simulink model "hdlcoder_addwc_eml"  (R2026a)
settings: Solver=FixedStepDiscrete  StopTime=10  FixedStep=1
settings Model: Creator=The MathWorks, Inc.  LastModifiedBy=The MathWorks, Inc.
settings OptimizationCC: ConditionallyExecuteInputs=off  InitFltsAndDblsToZero=on
settings DebuggingCC: AlgebraicLoopMsg=error  UnderspecifiedInitializationDetection=Classic  MultiTaskDSMMsg=warning  MultiTaskCondExecSysMsg=none  SingleTaskRateTransMsg=error
settings HardwareCC: ProdHWDeviceType=ASIC/FPGA
settings GRTTargetCC: TargetFcnLib=ansi_tfl_tmw_new.mat  CombineOutputUpdateFcns=off  GRTInterface=on

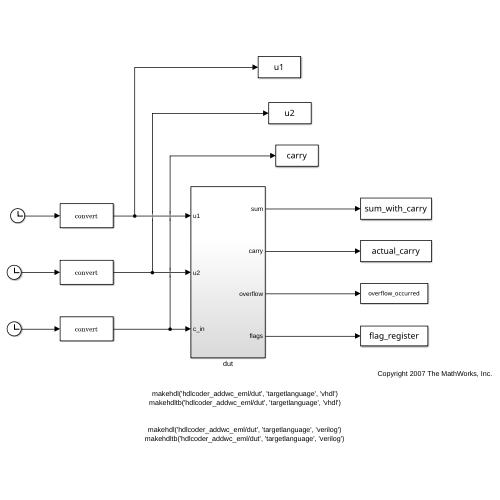
[thumbnail: Simulink's stored preview of the top-level diagram]
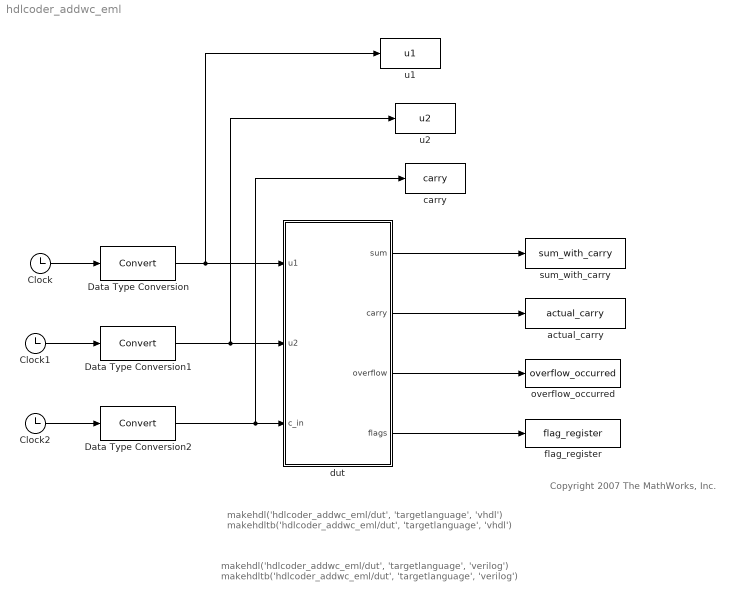
== system hdlcoder_addwc_eml ==
  note: Copyright 2007 The MathWorks, Inc.
  note: makehdl('hdlcoder_addwc_eml/dut', 'targetlanguage', 'vhdl')
      | makehdltb('hdlcoder_addwc_eml/dut', 'targetlanguage', 'vhdl')
  note: makehdl('hdlcoder_addwc_eml/dut', 'targetlanguage', 'verilog')
      | makehdltb('hdlcoder_addwc_eml/dut', 'targetlanguage', 'verilog')
  Clock : Clock
  Clock1 : Clock
  Clock2 : Clock
  Data Type Conversion : DataTypeConversion  SaturateOnIntegerOverflow=off  RndMeth=Floor
  Data Type Conversion1 : DataTypeConversion  SaturateOnIntegerOverflow=off  RndMeth=Floor
  Data Type Conversion2 : DataTypeConversion  SaturateOnIntegerOverflow=off  RndMeth=Floor
  actual_carry : ToWorkspace  VariableName=actual_carry  SampleTime=-1
  carry : ToWorkspace  VariableName=carry  SampleTime=-1
  dut : Subsystem
  flag_register : ToWorkspace  VariableName=flag_register  SampleTime=-1
  overflow_occurred : ToWorkspace  VariableName=overflow_occurred  SampleTime=-1
  sum_with_carry : ToWorkspace  VariableName=sum_with_carry  SampleTime=-1
  u1 : ToWorkspace  VariableName=u1  SampleTime=-1
  u2 : ToWorkspace  VariableName=u2  SampleTime=-1
  wires:
  Clock/1 -> Data Type Conversion/1
  Clock1/1 -> Data Type Conversion1/1
  Clock2/1 -> Data Type Conversion2/1
  Data Type Conversion/1 -> dut/1(u1), u1/1
  Data Type Conversion1/1 -> dut/2(u2), u2/1
  Data Type Conversion2/1 -> dut/3(c_in), carry/1
  dut/1(sum) -> sum_with_carry/1
  dut/2(carry) -> actual_carry/1
  dut/3(overflow) -> overflow_occurred/1
  dut/4(flags) -> flag_register/1

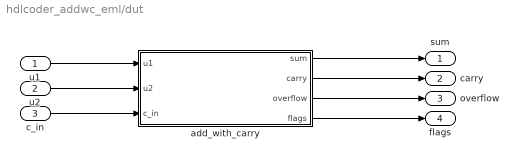
== system hdlcoder_addwc_eml/dut ==
  u1 : Inport
  u2 : Inport  Port=2
  c_in : Inport  Port=3
  add_with_carry : MATLAB Function  TreatAsAtomicUnit=on
  sum : Outport
  carry : Outport  Port=2
  overflow : Outport  Port=3
  flags : Outport  Port=4
  wires:
  add_with_carry/4(flags) -> flags/1
  c_in/1 -> add_with_carry/3(c_in)
  add_with_carry/3(overflow) -> overflow/1
  u2/1 -> add_with_carry/2(u2)
  add_with_carry/2(carry) -> carry/1
  u1/1 -> add_with_carry/1(u1)
  add_with_carry/1(sum) -> sum/1

== matlab function hdlcoder_addwc_eml/dut/add_with_carry ==
  settings: fimath=|
      | fimath(...
      | 'RoundMode', 'floor',...
      | 'OverflowMode', 'wrap',...
      | 'ProductMode', 'FullPrecision', 'ProductWordLength', 32,...
      | 'SumMode', 'FullPrecision', 'SumWordLength', 32,...
      | 'CastBeforeSum', true)
  data: u1 input fixdt(1,5,0); sum output; u2 input fixdt(1,5,0); carry output; overflow output; c_in input fixdt(0,1,0); flags output
function [sum,carry,overflow,flags] = fcn(u1,u2,c_in)
% add with carry
% also generates various CPU flags found in a FLAG regiser

nt_u1 = numerictype(u1);
fm_u1 = fimath(u1);

wlen  = nt_u1.WordLength;
ufix1_nt = numerictype(0, 1, 0);

% zero extend u1 by a bit
t_u1 = fi(u1, 1, wlen+1, 0);
t_u1 = bitset(t_u1, wlen+1, 0);

% zero extend u2 by a bit
t_u2 = fi(u2, 1, wlen+1, 0);
t_u2 = bitset(t_u2, wlen+1, 0);

% perform the addition
temp_sum = fi(t_u1+t_u2+c_in, 1, wlen+1, 0, fm_u1);

% Carry Flag (get msb)
carry = bitsliceget(temp_sum, wlen+1, wlen+1);

% Extract actual Sum
sum = fi(temp_sum, 1, wlen, 0, fm_u1);

% Negativity flag (N)
msb = getmsb(sum);

% Overflow Flag (V)
u1msb = getmsb(u1);
u2msb = getmsb(u2);
if((u1msb == u2msb) && (msb ~= u1msb))
    overflow = fi(1, ufix1_nt, fm_u1);
else
    overflow = fi(0, ufix1_nt, fm_u1);
end

if (all(sum))    
    zero = fi(1, 0, 1, 0);
else
    zero = fi(0, 0, 1, 0);
end

 
% construct the flag register
% flags = 'C N V Z'
flags = bitconcat(carry, msb, overflow, zero);
